simulink model "ssc_aircraft_elec_hybrid"  (R2025a)
settings: Solver=ode23t  StartTime=0.0  StopTime=FlightProfileLength  RelTol=1e-3  AbsTol=1e-3  EnableMultiTasking=on
PreLoadFcn:
  | ssc_aircraft_elec_default_params
PostLoadFcn:
  | warning('off','physmod:common:gl:sli:rtp:InvalidNonValueReference')
  | warning off Simulink:Engine:SortDiscontinuityInAlgLoop
model workspace (MATLAB code in the model file):
  | v0                 = 0; % Initial vehicle speed
  | wheel_radius = 0.15; % Wheel radius
  | k                   = 1e-2; % Motor losses (W/(N*M)^2)
  | t_torque        = 0.02; % Electric motor time constant
  | rpm0             = 2000; % Engine initial speed demand
undefined symbols (not defined in the file): Based, engine_ref_speed, gen_torque_demand, Height, motor_ref_speed
libraries: fl_lib x53, nesl_utility x31, ee_lib x9, ssc_aircraft_elec_lib x2, batteryecm_lib x1, simulink x1, sdl_lib x1, SimscapeFluids_lib x1
(part 1 of 2)
CloseFcn:
  | try,close(h1_ssc_aircraft_elec_hybrid),end
  | clear h1_ssc_aircraft_elec_hybrid
  | try,close(h2_ssc_aircraft_elec_hybrid),end
  | clear h2_ssc_aircraft_elec_hybrid
  | try,close(h3_ssc_aircraft_elec_hybrid),end
  | clear h3_ssc_aircraft_elec_hybrid
  | try,close(h4_ssc_aircraft_elec_hybrid),end
  | clear h4_ssc_aircraft_elec_hybrid
  | try,close(h5_ssc_aircraft_elec_hybrid),end
  | clear h5_ssc_aircraft_elec_hybrid
  | try,close(h6_ssc_aircraft_elec_hybrid),end
  | clear h6_ssc_aircraft_elec_hybrid
  | 
  | 
  | clear simlog_ssc_aircraft_elec_hybrid
  | clear logsout_ssc_aircraft_elec_hybrid
Description:
  | Hybrid Electric Aircraft Component Sizing
  | 
  | Copyright 2017-2025 The MathWorks, Inc.
settings Model: FPTRunName=Active  Creator=MathWorks  LastModifiedBy=smiller
settings SolverCC: AutoScaleAbsTol=off  AlgebraicLoopSolver=TrustRegion
settings DataIOCC: InitialState=xBaseline  LimitDataPoints=on  MaxDataPoints=10000  SaveOperatingPoint=on  SaveFormat=Array  ReturnWorkspaceOutputs=off  SignalLoggingName=simlog_ssc_aircraft_elec_hybrid
settings OptimizationCC: ReuseModelBlockBuffer=off  ExpressionDepthLimit=2147483647.0  LifeSpan=inf
settings DebuggingCC: AlgebraicLoopMsg=none  UnderspecifiedInitializationDetection=Classic  MergeDetectMultiDrivingBlocksExec=none  FcnCallInpInsideContextMsg=warning  UnconnectedInputMsg=warning  UnconnectedOutputMsg=warning  UnconnectedLineMsg=warning  StateNameClashWarn=warning  PregeneratedLibrarySubsystemCodeDiagnostic=none  SFUnexpectedBacktrackingDiag=warning  SFNoUnconditionalDefaultTransitionDiag=warning  SFExecutionAtInitializationDiag=none  ArithmeticOperatorsInVariantConditions=warning
settings HardwareCC: ProdBitPerPointer=32.0  ProdBitPerSizeT=32.0  ProdBitPerPtrDiffT=32.0  ProdLargestAtomicFloat=None  ProdIntDivRoundTo=Undefined  ProdEndianess=Unspecified  ProdWordSize=32.0  ProdHWDeviceType=32-bit Generic
settings ModelReferenceCC: EnableRefExpFcnMdlSchedulingChecks=on  PropagateSignalLabelsOutOfModel=off
settings SFSimCC: SimUseLocalCustomCode=off  CustomCodeUndefinedFunction=UseInterfaceOnly
settings RTWCC: RTWUseLocalCustomCode=off  GPUComputeCapability=3.5  DLArmComputeVersion=19.05
settings CodeAppCC: StateflowObjectComments=on
settings GRTTargetCC: TargetLangStandard=C89/C90 (ANSI)  CombineOutputUpdateFcns=off  GRTInterface=on
settings ConfigComp: CovMetricSettings=dw  CovSaveCumulativeToWorkspaceVar=on  CovSaveSingleToWorkspaceVar=on  CovExternalEMLEnable=off
settings SimscapeCC: SimscapeNormalizeSystem=off  SimscapeLogType=all  SimscapeLogSimulationStatistics=on  SimscapeLogName=simlog_ssc_aircraft_elec_hybrid  SimscapeLogDataHistory=10000.0

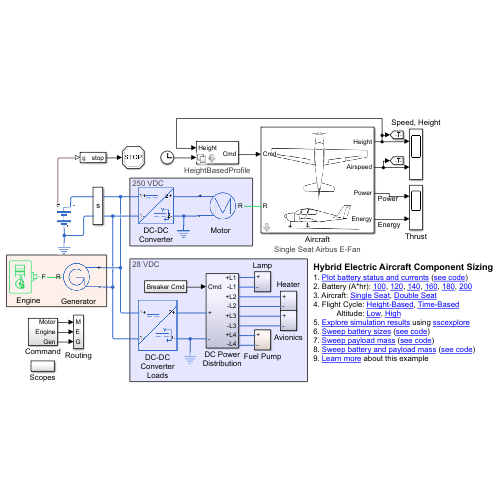
[thumbnail: Simulink's stored preview of the top-level diagram]
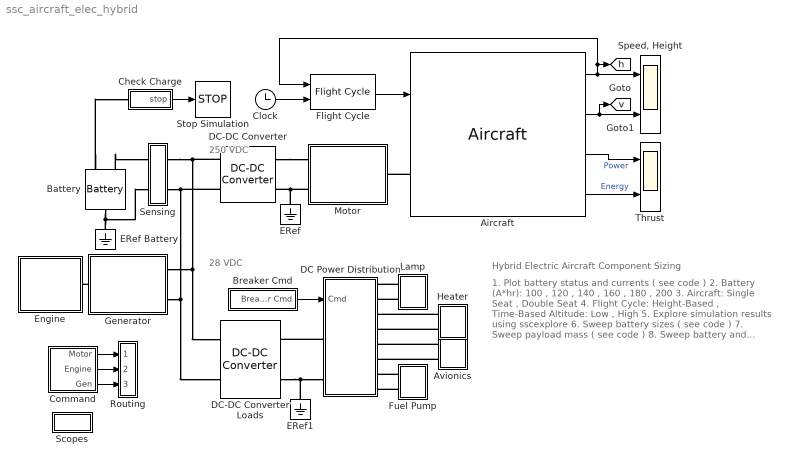
== system ssc_aircraft_elec_hybrid ==
  note: 250 VDC
  note: 28 VDC
  note: Hybrid Electric Aircraft Component Sizing
  note: 1. Plot battery status and currents ( see code )
      | 2. Battery (A*hr): 100 , 120 , 140 , 160 , 180 , 200
      | 3. Aircraft: Single Seat , Double Seat
      | 4. Flight Cycle: Height-Based , Time-Based
      | Altitude: Low , High
      | 5. Explore simulation results using sscexplore
      | 6. Sweep battery sizes ( see code )
      | 7. Sweep payload mass ( see code )
      | 8. Sweep battery and payload mass ( see code )
      | 9. Learn more about this example
  Aircraft : ssc_aircraft_elec_lib/Aircraft  Tag=PublishSubsystem  popup_aircraft_type=Single Seat Airbus E-Fan  aircraft_mass_cust=360  aircraft_wing_area_cust=10  aircraft_cl_cust=0.5  aircraft_cd_cust=0.05  battery_capacity=battery_capacity  battery_voltage=battery_vnom  battery_power_density=battery_pdensity  battery_mass=0  engine_system_mass=engine_system_mass  aircraft_max_thrust=max_thrust  aircraft_thrust_tau=thrust_tau  thrust_eff=thrust_eff  aircraft_h0=FlightProfileChoice.h0  aircraft_v0=0  earth_gravity=g_norm  checkbox_payload_mass=on  payload_mass=payload_mass
      settings: AttributesFormatString=%<popup_aircraft_type>
  Avionics : Subsystem
  Battery : batteryecm_lib/Battery  Vnom=201.6 V  prm_dir=1  R1_dis=2 Ohm  R1_ch=2 Ohm  R1=0.05 Ohm  prm_AH=2  AH=battery_capacity hr*A  V1=190 V  AH1=75 hr*A  prm_R2=1  R2=2000 Ohm  Tmeas=298.15 K  charge_measurement_port=simscape.enum.battery.enable.yes  prm_dyn=1  Rp1=0.005 Ohm  tau1=30 s  Rp2=0.005 Ohm  tau2=30 s  Rp3=0.005 Ohm  tau3=30 s  Rp4=0.005 Ohm  tau4=30 s  Rp5=0.005 Ohm  tau5=30 s  prm_fade=1  N_fade=100  AH_fade=45 hr*A  R1_fade=2.02 Ohm  R1_ch_fade=2.02 Ohm  V1_fade=10.35 V  prm_age=1  prm_age_OCV=1  OCV_age=0.9  SOC_age=60  Tmeas_age=298.15 K  delta_time_age_vec=[0] d  temperature_age_vec=[273] K  OCV_scaling_age=2.2134e6  OCV_offset_age=1.632e6  temp_exp_age=0.515833569 V  t_exp_age=0.75  Vnom_T2=12 V  R1_T2=2.2 Ohm  R1_T2_dis=2.2 Ohm  R1_T2_ch=2.2 Ohm  V1_T2=11.4 V  R2_T2=2200 Ohm  Rp1_T2=0.005 Ohm  tau1_T2=30 s  Rp2_T2=0.005 Ohm  tau2_T2=30 s  Rp3_T2=0.005 Ohm  tau3_T2=30 s  Rp4_T2=0.005 Ohm  tau4_T2=30 s  Rp5_T2=0.005 Ohm  tau5_T2=30 s  Tmeas2=273.15 K  thermal_port=simscape.enum.thermaleffects.omit  thermal_mass=30000 J/K  i_specify=off  i_priority=None  i=0 A  i_nominal_specify=off  i_nominal_value=1  i_nominal_unit=A  v_specify=off  v_priority=None  v=0 V  v_nominal_specify=off  v_nominal_value=1  v_nominal_unit=V  charge_specify=on  charge_priority=High  charge=battery_capacity hr*A  charge_nominal_specify=off  charge_nominal_value=1  charge_nominal_unit=A*hr  num_cycles_specify=off  num_cycles_priority=High  num_cycles=0  num_cycles_nominal_specify=off  num_cycles_nominal_value=1  num_cycles_nominal_unit=1  temperature_specify=off  temperature_priority=High  temperature=298.15 K  temperature_nominal_specify=off  temperature_nominal_value=1  temperature_nominal_unit=K
      settings: InternalSimscapePortConfiguration="{\"Bottom\":[],\"Left\":[{\"id\":\"p\",\"label\":\"+\",\"type\":\"foundation.electrical.electrical\"},{\"id\":\"q\",\"label\":\"q\",\"type\":\"output\"}],\"Right\":[{\"id\":\"n\",\"label\":\"-\",\"type\":\"foundation.electrical.electrical\"}],\"Top\":[]}"
  Breaker Cmd : Subsystem
  Check Charge : Subsystem  mask{q_battery_limit=20}
      mask prompts: q_battery_limit "Battery charge lower limit (A*hr)"
  Clock : Clock
  Command : Subsystem
  DC Power Distribution : Subsystem  Tag=PublishSubsystem
  DC-DC Converter : ee_lib/Semiconductors & Converters/Converters/DC-DC Converter  Vref_option=ee.enum.converters.voltageref.internal  v_ref=250 V  P_rated=200 kW  droop_enabled=true  droop_param=ee.enum.converters.droop.value  droop=0.001 V/A  droop_percent=2  Vref_droop=10 V  reversible=ee.enum.converters.directionality.bidirectional  G_diode=1e-8 1/Ohm  P_fixed=100 W  losses_option=ee.enum.converters.lossesOption.proportionalToSquaredCurrent  eff_rated=97  tableOption=ee.enum.converters.lossTableOption.current  i_eff_vec=[1, 2, 3, 4] A  v_eff_vec=[15, 30, 45] V  eff_vec=[90, 80, 70, 60]  eff_2D_table=[90, 85, 80; 80, 75, 70; 70, 65, 60; 60, 55, 50]  model_dynamics=ee.enum.converters.dynamics.yes  tau=0.02 s  v_ini=250 V  v1_min=1 V  R1=1000 Ohm  R2=1000 Ohm  fault_condition=ee.enum.faults.faultInputCondition.greaterThan  fault_threshold=0.5  T_eff_vec=[280, 300, 320] K  eff_3D_table=repmat([66; 76; 80; 74], 1, 3, 3)  thermal_mass=100 J/K  initial_temperature=298.15 K
      settings: InternalSimscapePortConfiguration="{\"Bottom\":[],\"Left\":[{\"id\":\"p1\",\"label\":\"1+\",\"type\":\"foundation.electrical.electrical\"},{\"id\":\"n1\",\"label\":\"1-\",\"type\":\"foundation.electrical.electrical\"}],\"Right\":[{\"id\":\"p2\",\"label\":\"2+\",\"type\":\"foundation.electrical.electrical\"},{\"id\":\"n2\",\"label\":\"2-\",\"type\":\"foundation.electrical.electrical\"}],\"Top\":[]}"
  DC-DC Converter Loads : ee_lib/Semiconductors & Converters/Converters/DC-DC Converter  Vref_option=ee.enum.converters.voltageref.internal  v_ref=28 V  P_rated=4 kW  droop_enabled=true  droop_param=ee.enum.converters.droop.value  droop=0.01 V/A  droop_percent=2  Vref_droop=10 V  reversible=ee.enum.converters.directionality.unidirectional  G_diode=1e-8 1/Ohm  P_fixed=100 W  losses_option=ee.enum.converters.lossesOption.proportionalToSquaredCurrent  eff_rated=97  tableOption=ee.enum.converters.lossTableOption.current  i_eff_vec=[1, 2, 3, 4] A  v_eff_vec=[15, 30, 45] V  eff_vec=[90, 80, 70, 60]  eff_2D_table=[90, 85, 80; 80, 75, 70; 70, 65, 60; 60, 55, 50]  model_dynamics=ee.enum.converters.dynamics.yes  tau=0.02 s  v_ini=28 V  v1_min=1 V  R1=1000 Ohm  R2=1000 Ohm  fault_condition=ee.enum.faults.faultInputCondition.greaterThan  fault_threshold=0.5  T_eff_vec=[280, 300, 320] K  eff_3D_table=repmat([66; 76; 80; 74], 1, 3, 3)  thermal_mass=100 J/K  initial_temperature=298.15 K
      settings: InternalSimscapePortConfiguration="{\"Bottom\":[],\"Left\":[{\"id\":\"p1\",\"label\":\"1+\",\"type\":\"foundation.electrical.electrical\"},{\"id\":\"n1\",\"label\":\"1-\",\"type\":\"foundation.electrical.electrical\"}],\"Right\":[{\"id\":\"p2\",\"label\":\"2+\",\"type\":\"foundation.electrical.electrical\"},{\"id\":\"n2\",\"label\":\"2-\",\"type\":\"foundation.electrical.electrical\"}],\"Top\":[]}"
  ERef : fl_lib/Electrical/Electrical Elements/Electrical Reference
  ERef Battery : fl_lib/Electrical/Electrical Elements/Electrical Reference
  ERef1 : fl_lib/Electrical/Electrical Elements/Electrical Reference
  Engine : Subsystem
      mask Display:
      | image('Driveline_Engine_IMAGE.png');
      | %{
      | patch([0 374 374 0 0],[183 40 40 183 183],[1 1 1]);
      | plot([200.294537656123;201.704177092068;202.879954177142;203.81054553527;204.486989062962;204.902770239264;205.053884864158;204.938877621199;204.558856093007;203.917480094638;203.02092642757;201.877829393721;200.499197642409;198.898308151034;197.090578360535;195.093417696999;192.926059909376;191.349221415216], [79.0962651705123;81.4129472419303;83.856642682368;86.4038173688741;89.0299406167901;91.7097214236537;94.4173520353776;97.1267564890293;99.8118417386092;102.446748945347;105.006102512455;107.465254465996;109.80052182835;111.989414698229;114.010852840726;115.845368701499;117.475294889959;118.468271604945])
      | plot([180.070315486255;177.215173525063;174.340173090774;171.473002009205;168.641272705228;165.872256280019;163.192619875453;160.628169854943;158.203603274058;155.942270034374;153.865948011161;151.994633320535;150.346347745932;148.936965178479;147.780058742747;146.886770080143;146.265702048809;145.922835873396;145.861473542603;146.08220600922;146.58290749893;147.358755982674;148.402279615432;149.703428694174;151.249672441989;153.026119686324;155.015662269112;157.199139807684;159.555524219735;162.062122235246;164.694793945081;167.42818528151;170.23597219174;173.091114152932;175.966114587221;178.83328566879;181.665014972767;184.434031397976;185.486929355725], [123.25590763568;123.598773811093;123.660136141886;123.439403675268;122.938702185559;122.162853701815;121.119330069056;119.818180990315;118.2719372425;116.495489998164;114.505947415377;112.322469876805;109.966085464754;107.459487449243;104.826815739408;102.093424402979;99.2856374927491;96.4304955315569;93.5554950972677;90.688324015699;87.8565947117214;85.0875782865128;82.4079418819464;79.8434918614364;77.4189252805513;75.1575920408679;73.081270017655;71.2099553270291;69.5616697524256;68.1522871849724;66.9953807492411;66.1020920866371;65.4810240553025;65.1381578798894;65.0767955490969;65.2975280157144;65.7982295054238;66.5740779891678;66.9481130562871])
      | plot([182.088349247351;182.056804583223;181.962474383197;181.806267098667;181.589687091173;181.314820144583;180.98431337785;180.601349751811;180.169617415534;179.693274187426;179.176907513169;178.625490286111;178.044332955585;177.439032384376;176.815417947876;176.17949539401;175.537389004603;174.895282615196;174.25936006133;173.63574562483;173.030445053621;172.449287723095;171.897870496037;171.38150382178;170.905160593672;170.473428257395;170.090464631356;169.759957864623;169.485090918033;169.268510910539;169.112303626009;169.017973425983;168.986428761855;169.017973425983;169.112303626009;169.268510910539;169.485090918033;169.759957864623;170.090464631356;170.473428257395;170.905160593672;171.38150382178;171.897870496037;172.449287723095;173.030445053621;173.63574562483;174.25936006133;174.895282615196;175.537389004603;176.17949539401;176.815417947876;177.439032384376;178.044332955585;178.625490286111;179.176907513169;179.693274187426;180.169617415534;180.601349751811;180.98431337785;181.314820144583;181.589687091173;181.806267098667;181.962474383197;182.056804583223;182.088349247351;182.088349247351], [94.3432759959251;93.7073437064164;93.0775357924916;92.4599176486499;91.8604372752408;91.2848679959696;90.7387528576339;90.2273512475527;89.7555882427917;89.3280071789786;88.9487258954975;88.6213970784445;88.3491730832641;88.1346755758426;87.9799702844327;87.8865471055612;87.8553057555109;87.8865471055612;87.9799702844327;88.1346755758426;88.3491730832641;88.6213970784445;88.9487258954975;89.3280071789786;89.7555882427917;90.2273512475527;90.7387528576339;91.2848679959696;91.8604372752408;92.4599176486499;93.0775357924916;93.7073437064164;94.3432759959251;94.9792082854337;95.6090161993586;96.2266343432003;96.8261147166093;97.4016839958805;97.9477991342162;98.4592007442974;98.9309637490584;99.3585448128716;99.7378260963527;100.065154913406;100.337378908586;100.551876416008;100.706581707417;100.800004886289;100.831246236339;100.800004886289;100.706581707417;100.551876416008;100.337378908586;100.065154913406;99.7378260963526;99.3585448128716;98.9309637490584;98.4592007442974;97.9477991342162;97.4016839958805;96.8261147166093;96.2266343432003;95.6090161993586;94.9792082854338;94.3432759959251;94.3432759959251])
      | plot([201.615249970928;201.583705306799;201.489375106774;201.333167822243;201.11658781475;200.84172086816;200.511214101427;200.128250475388;199.69651813911;199.220174911002;198.703808236745;198.152391009688;197.571233679162;196.965933107953;196.342318671452;195.706396117586;195.06428972818;194.422183338773;193.786260784907;193.162646348407;192.557345777197;191.976188446671;191.424771219614;190.908404545357;190.432061317249;190.000328980971;189.617365354932;189.286858588199;189.011991641609;188.795411634116;188.639204349585;188.54487414956;188.513329485431;188.54487414956;188.639204349585;188.795411634116;189.011991641609;189.286858588199;189.617365354932;190.000328980971;190.432061317249;190.908404545357;191.424771219614;191.976188446671;192.557345777197;193.162646348407;193.786260784907;194.422183338773;195.06428972818;195.706396117586;196.342318671452;196.965933107953;197.571233679162;198.152391009688;198.703808236745;199.220174911002;199.69651813911;200.128250475388;200.511214101427;200.84172086816;201.11658781475;201.333167822243;201.489375106774;201.583705306799;201.615249970928;201.615249970928], [74.7533852700144;74.1174529805057;73.487645066581;72.8700269227392;72.2705465493302;71.694977270059;71.1488621317233;70.6374605216421;70.165697516881;69.7381164530679;69.3588351695868;69.0315063525339;68.7592823573535;68.5447848499319;68.390079558522;68.2966563796505;68.2654150296003;68.2966563796505;68.390079558522;68.5447848499319;68.7592823573535;69.0315063525339;69.3588351695868;69.7381164530679;70.165697516881;70.6374605216421;71.1488621317233;71.694977270059;72.2705465493302;72.8700269227392;73.487645066581;74.1174529805057;74.7533852700144;75.3893175595231;76.0191254734479;76.6367436172896;77.2362239906986;77.8117932699698;78.3579084083055;78.8693100183867;79.3410730231478;79.7686540869609;80.147935370442;80.4752641874949;80.7474881826754;80.9619856900969;81.1166909815068;81.2101141603783;81.2413555104285;81.2101141603783;81.1166909815068;80.9619856900969;80.7474881826753;80.4752641874949;80.147935370442;79.7686540869609;79.3410730231478;78.8693100183867;78.3579084083055;77.8117932699698;77.2362239906986;76.6367436172896;76.0191254734479;75.3893175595231;74.7533852700145;74.7533852700144])
      | plot([201.615249970928;201.583705306799;201.489375106774;201.333167822243;201.11658781475;200.84172086816;200.511214101427;200.128250475388;199.69651813911;199.220174911002;198.703808236745;198.152391009688;197.571233679162;196.965933107953;196.342318671452;195.706396117586;195.06428972818;194.422183338773;193.786260784907;193.162646348407;192.557345777197;191.976188446671;191.424771219614;190.908404545357;190.432061317249;190.000328980971;189.617365354932;189.286858588199;189.011991641609;188.795411634116;188.639204349585;188.54487414956;188.513329485431;188.54487414956;188.639204349585;188.795411634116;189.011991641609;189.286858588199;189.617365354932;190.000328980971;190.432061317249;190.908404545357;191.424771219614;191.976188446671;192.557345777197;193.162646348407;193.786260784907;194.422183338773;195.06428972818;195.706396117586;196.342318671452;196.965933107953;197.571233679162;198.152391009688;198.703808236745;199.220174911002;199.69651813911;200.128250475388;200.511214101427;200.84172086816;201.11658781475;201.333167822243;201.489375106774;201.583705306799;201.615249970928;201.615249970928], [74.7533852700144;74.1174529805057;73.487645066581;72.8700269227392;72.2705465493302;71.694977270059;71.1488621317233;70.6374605216421;70.165697516881;69.7381164530679;69.3588351695868;69.0315063525339;68.7592823573535;68.5447848499319;68.390079558522;68.2966563796505;68.2654150296003;68.2966563796505;68.390079558522;68.5447848499319;68.7592823573535;69.0315063525339;69.3588351695868;69.7381164530679;70.165697516881;70.6374605216421;71.1488621317233;71.694977270059;72.2705465493302;72.8700269227392;73.487645066581;74.1174529805057;74.7533852700144;75.3893175595231;76.0191254734479;76.6367436172896;77.2362239906986;77.8117932699698;78.3579084083055;78.8693100183867;79.3410730231478;79.7686540869609;80.147935370442;80.4752641874949;80.7474881826754;80.9619856900969;81.1166909815068;81.2101141603783;81.2413555104285;81.2101141603783;81.1166909815068;80.9619856900969;80.7474881826753;80.4752641874949;80.147935370442;79.7686540869609;79.3410730231478;78.8693100183867;78.3579084083055;77.8117932699698;77.2362239906986;76.6367436172896;76.0191254734479;75.3893175595231;74.7533852700145;74.7533852700144])
      | plot([142.90856779553;142.90856779553;208.103220211342;208.103220211342], [139.948037685826;218.181620584801;218.181620584801;139.948037685826])
      | plot([142.90856779553;208.103220211342], [179.064829135314;179.064829135314])
      | plot([149.459528038278;149.459528038278], [179.064829135314;172.576858894899])
      | plot([201.615249970928;201.615249970928], [179.064829135314;172.576858894899])
      | plot([142.90856779553;208.103220211342;208.103220211342;142.90856779553;142.90856779553], [179.064829135314;179.064829135314;152.986968168989;152.986968168989;179.064829135314])
      | plot([142.90856779553;208.103220211342], [192.103759618476;192.103759618476])
      | plot([180.639579193667;200.229469919577], [99.0045361686498;79.4776354450732])
      | plot([173.332738922909;192.92262964882], [87.8553057555109;68.3284050319344])
      | plot([183.663099305704;200.481429928914], [153.553878189996;76.9580353517085])
      | plot([184.544959338382;174.970478983596], [95.0361660216004;153.553878189996])
      | plot([183.474129298702;186.749609420076;206.654450157657;201.615249970928;197.961829835549], [76.9580353517085;62.0923948008567;67.8874750155956;88.1702557671815;87.7923157531768])
      | plot([164.199188584462;187.694459455088], [94.7842060122639;95.1621460262686])
      | plot([175.537389004603;175.285428995267], [106.50034644641;81.9342455361038])
      | plot([142.90856779553;208.103220211342], [172.576858894899;172.576858894899])
      | plot([297.86397353746;317.389525743201], [71.0999651346356;71.0999651346356]+60)
      | plot([269.518472487107;297.86397353746;297.86397353746;269.518472487107;269.518472487107], [85.2727156598121;85.2727156598121;56.927214609459;56.927214609459;85.2727156598121]+60)
      | plot([258.180272066966;269.518472487107;269.518472487107;258.180272066966], [42.7544640842825;42.7544640842825;99.4454661849886;99.4454661849886]+60)
      | plot([108.893966535106;108.245686045801;107.603648851995;106.974038122836;106.362917353826;105.776171972045;105.219452656266;104.698120917834;104.217197466378;103.781313857637;103.394667889039;103.060983172626;102.783473274627;102.564810767061;102.40710148941;102.31186426823;102.280016290024;102.280016290024;102.31186426823;102.40710148941;102.564810767061;102.783473274627;103.060983172626;103.394667889039;103.781313857637;104.217197466378;104.698120917834;105.219452656266;105.776171972045;106.362917353826;106.974038122836;107.603648851995;108.245686045801;108.893966535106;249.67662175186;250.324902241165;250.966939434972;251.596550164131;252.20767093314;252.794416314921;253.3511356307;253.872467369133;254.353390820588;254.78927442933;255.175920397927;255.50960511434;255.787115012339;256.005777519905;256.163486797556;256.258724018736;256.290571996942;256.290571996942;256.258724018736;256.163486797556;256.005777519905;255.787115012339;255.50960511434;255.175920397927;254.78927442933;254.353390820588;253.872467369133;253.3511356307;252.794416314921;252.20767093314;251.596550164131;250.966939434972;250.324902241165;249.67662175186;108.893966535106], [233.173241140321;233.141393162114;233.046155940935;232.888446663284;232.669784155718;232.392274257719;232.058589541306;231.671943572708;231.236059963967;230.755136512511;230.233804774079;229.6770854583;229.090340076519;228.479219307509;227.84960857835;227.207571384544;226.559290895239;46.5338642243296;45.8855837350246;45.2435465412178;44.6139358120588;44.0028150430496;43.4160696612682;42.8593503454891;42.3380186070568;41.8570951556014;41.4212115468599;41.0345655782626;40.7008808618494;40.42337096385;40.2047084562844;40.0469991786335;39.9517619574538;39.9199139792472;39.9199139792472;39.9517619574538;40.0469991786335;40.2047084562844;40.42337096385;40.7008808618494;41.0345655782626;41.4212115468599;41.8570951556014;42.3380186070568;42.8593503454891;43.4160696612682;44.0028150430496;44.6139358120588;45.2435465412178;45.8855837350246;46.5338642243296;226.559290895239;227.207571384544;227.84960857835;228.479219307509;229.090340076519;229.6770854583;230.233804774079;230.755136512511;231.236059963967;231.671943572708;232.058589541306;232.392274257719;232.669784155718;232.888446663284;233.046155940935;233.141393162114;233.173241140321;233.173241140321])
      | %}
  Flight Cycle : ssc_aircraft_elec_lib/Flight Cycle  popup_flight_cycle_type=Height-Based  flight_cycle_max_height=FlightProfileChoice.FlightProfileHeight  flight_cycle_ascent_start_time=FlightProfileChoice.LevelFlightTime  flight_cycle_duration=FlightProfileChoice.FlightProfileLength  flight_cycle_ascent_duration=FlightProfileChoice.ClimbFlightTime
      settings: AttributesFormatString=%<ActiveVariant>
  Fuel Pump : Subsystem  Tag=PublishSubsystem
  Generator : Subsystem  Tag=PublishSubsystem
      mask Display:
      | image('Generator_IMAGE.png');
      | % Circle
      | %{
      | plot(sin(0:0.1:2.2*pi)*0.9,cos(0:0.1:2.2*pi)*0.9);
      | 
      | % In/out
      | plot([-1.5 -0.9],[0 0]);
      | plot([1.5 0.58],[1 1]*0.65);
      | plot([1.5 0.55],-[1 1]*0.68);
      | 
      | % 'M'
      | %plot([0.5 0.5],[-0.5 0.5]);
      | %plot([-0.5 -0.5],[-0.5 0.5]);
      | %plot([0.5 0],[0.5 -0.5]);
      | %plot([-0.5 0],[0.5 -0.5]);
      | 
      | % 'G'
      | plot(sin(0.5:-0.1:-1.5*pi)*0.5,cos(-0.5:0.1:1.5*pi)*0.5);
      | plot([0 0.5 0.5],[0 0 -0.5]);
      | 
      | % Plot points to set plot range
      | color('white');plot(1.9,1.2);plot(-1.9,-1.2)
      | color('black');
      | %}
  Heater : Subsystem
  Lamp : Subsystem
  Motor : Subsystem  Tag=PublishSubsystem
      mask Display: image('Motor_IMAGE.png');
  Routing : Subsystem
  Scopes : Subsystem
  Sensing : Subsystem
      mask Display: disp('s');
  "Speed, Height" : Scope  NumInputPorts=2
      settings: ActiveDisplayYMinimum=-12.5  ActiveDisplayYMaximum=1112.5
  Stop Simulation : Stop
  Thrust : Scope  NumInputPorts=2
      settings: ActiveDisplayYMinimum=13.58364  ActiveDisplayYMaximum=68.87509  DataLoggingMaxPoints=50000  DataLoggingVariableName=ScopeData6
  tag scope: h=global, v=global
  wires:
  Command/1(Motor) -> Routing/1(M)
  Aircraft/2 -> [v], "Speed, Height"/2
  Aircraft/3 -> Thrust/1  "Power"
  Aircraft/4 -> Thrust/2  "Energy"
  Command/2(Engine) -> Routing/2(E)
  Command/3(Gen) -> Routing/3(G)
  Clock/1 -> Flight Cycle/2
  Aircraft/1 -> [h], Flight Cycle/1, "Speed, Height"/1
  Flight Cycle/1 -> Aircraft/1
  Check Charge/1(stop) -> Stop Simulation/1
  Breaker Cmd/1(Breaker Cmd) -> DC Power Distribution/1(Cmd)
  connections:
  Aircraft/LConn1 -- Motor/LConn1
  DC-DC Converter/RConn1 -- Motor/RConn1
  DC Power Distribution/LConn1 -- DC-DC Converter Loads/RConn1
  Heater/LConn1 -- DC Power Distribution/RConn3
  Lamp/LConn2 -- DC Power Distribution/RConn2
  Lamp/LConn1 -- DC Power Distribution/RConn1
  Heater/LConn2 -- DC Power Distribution/RConn4
  DC-DC Converter Loads/RConn2 -- DC Power Distribution/LConn2 -- ERef1/LConn1
  ERef/LConn1 -- Motor/RConn2 -- DC-DC Converter/RConn2
  DC-DC Converter/LConn1 -- Generator/RConn1 -- DC-DC Converter Loads/LConn1 -- Sensing/RConn1
  Sensing/RConn2 -- DC-DC Converter/LConn2 -- Generator/RConn2 -- DC-DC Converter Loads/LConn2
  Avionics/LConn1 -- DC Power Distribution/RConn5
  Avionics/LConn2 -- DC Power Distribution/RConn6
  Generator/LConn1 -- Engine/RConn1
  Fuel Pump/LConn1 -- DC Power Distribution/RConn7
  Fuel Pump/LConn2 -- DC Power Distribution/RConn8
  Battery/LConn2 -- Check Charge/LConn1
  Battery/LConn1 -- Sensing/LConn1
  Battery/RConn1 -- ERef Battery/LConn1 -- Sensing/LConn2

== system ssc_aircraft_elec_hybrid/Avionics ==
  Electrical Power : Subsystem
  Resistor : fl_lib/Electrical/Electrical Elements/Resistor  R=1.5 Ohm  i_specify=off  i_priority=None  i=0 A  i_nominal_specify=off  i_nominal_value=1  i_nominal_unit=A  v_specify=off  v_priority=None  v=0 V  v_nominal_specify=off  v_nominal_value=1  v_nominal_unit=V
  + : PMIOPort  Side=Left
  - : PMIOPort  Port=2  Side=Left
  connections:
  Electrical Power/LConn1 -- +/RConn1
  Resistor/LConn1 -- Electrical Power/RConn1
  Electrical Power/LConn2 -- Resistor/RConn1 -- -/RConn1

== system ssc_aircraft_elec_hybrid/Breaker Cmd ==
  Avionics Breaker : Constant
  Fuel Pump Breaker : Constant
  Heater Breaker OFF : Constant  Value=0
  Heater Breaker ON : Constant
  Lamp Breaker : Constant
  Mux : Mux
  Switch : Switch  Threshold=800  SaturateOnIntegerOverflow=off  InputSameDT=off
  Breaker Cmd : Outport  VectorParamsAs1DForOutWhenUnconnected=off
  wires:
  Fuel Pump Breaker/1 -> Mux/4
  Lamp Breaker/1 -> Mux/1
  Avionics Breaker/1 -> Mux/3
  Switch/1 -> Mux/2
  Mux/1 -> Breaker Cmd/1
  Heater Breaker OFF/1 -> Switch/3
  [h] -> Switch/2
  Heater Breaker ON/1 -> Switch/1

== system ssc_aircraft_elec_hybrid/Check Charge ==
  Compare To Constant : simulink/Logic and Bit Operations/Compare To Constant  relop=<=  const=q_battery_limit  OutDataTypeStr=boolean
  PS-Simulink Converter : nesl_utility/PS-Simulink Converter  PhysicalDomain=network_engine_domain  SubClassName=ps_output  LeftPortType=input  RightPortType=output  PseudoPeriodic=off  Frequencies=[]  VectorFormat=1-D array  Unit=A*hr  AffineConversion=off
  q : PMIOPort  Side=Left
  stop : Outport  VectorParamsAs1DForOutWhenUnconnected=off
  tag scope: Chg_battery=global
  wires:
  PS-Simulink Converter/1 -> [Chg_battery], Compare To Constant/1
  Compare To Constant/1 -> stop/1
  connections:
  q/RConn1 -- PS-Simulink Converter/LConn1

== system ssc_aircraft_elec_hybrid/Command ==
  Engine RPM demand : Constant  Value=engine_ref_speed
  Gain : Gain  Gain=-1
  Generator torque demand : Constant  Value=gen_torque_demand
  Ref RPM : Constant  Value=motor_ref_speed
  Steady-state correction factor as proportional-only control : Gain  Gain=1.08
  Motor : Outport  VectorParamsAs1DForOutWhenUnconnected=off
  Engine : Outport  Port=2  VectorParamsAs1DForOutWhenUnconnected=off
  Gen : Outport  Port=3  VectorParamsAs1DForOutWhenUnconnected=off
  wires:
  Ref RPM/1 -> Motor/1
  Generator torque demand/1 -> Gain/1
  Steady-state correction factor as proportional-only control/1 -> Engine/1
  Engine RPM demand/1 -> Steady-state correction factor as proportional-only control/1
  Gain/1 -> Gen/1

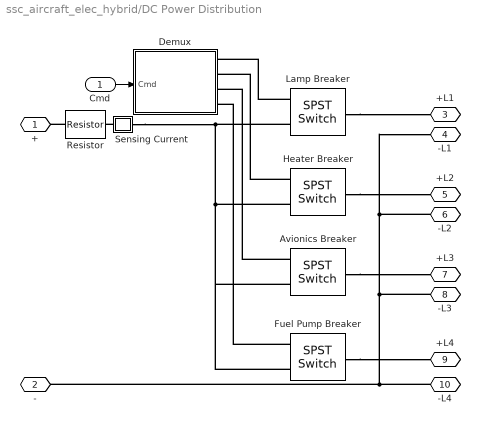
== system ssc_aircraft_elec_hybrid/DC Power Distribution ==
  Cmd : Inport
  Avionics Breaker : ee_lib/Switches & Breakers/SPST Switch  R_closed=0.001 Ohm  G_open=1e-3 S  Threshold=0.5 V  Width=0 V  model_dynamics=0  t_on=1e-3 s  t_off=1e-3 s  initial_vT=0 V
      settings: InternalSimscapePortConfiguration="{\"Bottom\":[],\"Left\":[{\"id\":\"vT\",\"label\":\"vT\",\"type\":\"input\"},{\"id\":\"p\",\"label\":\"\",\"type\":\"foundation.electrical.electrical\"}],\"Right\":[{\"id\":\"n\",\"label\":\"\",\"type\":\"foundation.electrical.electrical\"}],\"Top\":[]}"
  Demux : Subsystem
  Fuel Pump Breaker : ee_lib/Switches & Breakers/SPST Switch  R_closed=0.001 Ohm  G_open=1e-3 S  Threshold=0.5 V  Width=0 V  model_dynamics=0  t_on=1e-3 s  t_off=1e-3 s  initial_vT=0 V
      settings: InternalSimscapePortConfiguration="{\"Bottom\":[],\"Left\":[{\"id\":\"vT\",\"label\":\"vT\",\"type\":\"input\"},{\"id\":\"p\",\"label\":\"\",\"type\":\"foundation.electrical.electrical\"}],\"Right\":[{\"id\":\"n\",\"label\":\"\",\"type\":\"foundation.electrical.electrical\"}],\"Top\":[]}"
  Heater Breaker : ee_lib/Switches & Breakers/SPST Switch  R_closed=0.001 Ohm  G_open=1e-3 S  Threshold=0.5 V  Width=0 V  model_dynamics=0  t_on=1e-3 s  t_off=1e-3 s  initial_vT=0 V
      settings: InternalSimscapePortConfiguration="{\"Bottom\":[],\"Left\":[{\"id\":\"vT\",\"label\":\"vT\",\"type\":\"input\"},{\"id\":\"p\",\"label\":\"\",\"type\":\"foundation.electrical.electrical\"}],\"Right\":[{\"id\":\"n\",\"label\":\"\",\"type\":\"foundation.electrical.electrical\"}],\"Top\":[]}"
  Lamp Breaker : ee_lib/Switches & Breakers/SPST Switch  R_closed=0.001 Ohm  G_open=1e-3 S  Threshold=0.5 V  Width=0 V  model_dynamics=0  t_on=1e-3 s  t_off=1e-3 s  initial_vT=0 V
      settings: InternalSimscapePortConfiguration="{\"Bottom\":[],\"Left\":[{\"id\":\"vT\",\"label\":\"vT\",\"type\":\"input\"},{\"id\":\"p\",\"label\":\"\",\"type\":\"foundation.electrical.electrical\"}],\"Right\":[{\"id\":\"n\",\"label\":\"\",\"type\":\"foundation.electrical.electrical\"}],\"Top\":[]}"
  Resistor : fl_lib/Electrical/Electrical Elements/Resistor  R=0.002 Ohm  i_specify=off  i_priority=None  i=0 A  i_nominal_specify=off  i_nominal_value=1  i_nominal_unit=A  v_specify=off  v_priority=None  v=0 V  v_nominal_specify=off  v_nominal_value=1  v_nominal_unit=V
  Sensing Current : Subsystem
      mask Display: disp('i')
  + : PMIOPort  Side=Left
  - : PMIOPort  Port=2  Side=Left
  +L1 : PMIOPort  Port=3  Side=Right
  -L1 : PMIOPort  Port=4  Side=Right
  +L2 : PMIOPort  Port=5  Side=Right
  -L2 : PMIOPort  Port=6  Side=Right
  +L3 : PMIOPort  Port=7  Side=Right
  -L3 : PMIOPort  Port=8  Side=Right
  +L4 : PMIOPort  Port=9  Side=Right
  -L4 : PMIOPort  Port=10  Side=Right
  wires:
  Cmd/1 -> Demux/1(Cmd)
  connections:
  -L4/RConn1 -- -L1/RConn1 -- -L2/RConn1 -- -L3/RConn1 -- -/RConn1
  Lamp Breaker/RConn1 -- +L1/RConn1
  Heater Breaker/RConn1 -- +L2/RConn1
  Avionics Breaker/RConn1 -- +L3/RConn1
  Fuel Pump Breaker/RConn1 -- +L4/RConn1
  Resistor/LConn1 -- +/RConn1
  Lamp Breaker/LConn1 -- Demux/RConn1
  Heater Breaker/LConn1 -- Demux/RConn2
  Avionics Breaker/LConn1 -- Demux/RConn3
  Fuel Pump Breaker/LConn1 -- Demux/RConn4
  Fuel Pump Breaker/LConn2 -- Avionics Breaker/LConn2 -- Heater Breaker/LConn2 -- Lamp Breaker/LConn2 -- Sensing Current/RConn1
  Sensing Current/LConn1 -- Resistor/RConn1

== system ssc_aircraft_elec_hybrid/Engine ==
  Engine : sdl_lib/Engines & Motors/Generic Engine  input_type=sdl.enum.GenericEngineInputType.NormalizedThrottle  model_parameterization=1  engine_type=1  Trq_max=380 N*m  w_Trq_max=4300 rpm  P_max=50e3 W  w_P_max=5500 rpm  w_max=7000 rpm  w_min=500 rpm  w_tab=[ 500 1000 2e+3 3e+3 4e+3 5e+3 6e+3 7e+3 ] rpm  trq_tab=[ 380 380 380 380 350 280 200 80 ] N*m  pwr_tab=[ 2e+4 4e+4 7.8e+4 1.2e+5 1.45e+5 1.48e+5 1.25e+5 6e+4 ] W  interp_method=1  w_thr=20 rpm  model_inertia=1  inertia=0.2 kg*m^2  initial_velocity=2000 rpm  model_time_constant=1  time_constant=0.2 s  initial_normalized_throttle=0.15  fc_model=4  fc_per_rev=25 mg/rev  fc_w_tab=[ 1000 2e+3 3e+3 4e+3 5e+3 6e+3 ] rpm  fc_trq_tab=[ 0 80 160 200 240 320 360 400 ] N*m  fc_tab=[ 0.5 0.9 1.4 1.6 1.9 2.7 3.4 4.4; 1 1.7 2.7 3.1 3.6 5 6 7.4; 1.4 2.7 4 4.8 5.6 7.5 8.5 10.5; 2 3.6 5.8 6.7 8 10.4 11.7 13.3; 2.5 4.8 7.9 9.4 10.8 14 16.2 18.6; 3.1 6 10.3 11.9 13.8 18.4 22 26.5 ] g/s  bmep_tab=[ 0 250 500 625 750 1000 1.15e+3 1.25e+3 ] kPa  bsfc_tab=[ 410 380 300 280 270 290 320 380; 410 370 290 270 260 270 285 320; 415 380 290 275 265 270 270 300; 420 390 310 290 285 280 280 285; 430 410 340 320 310 300 310 320; 450 430 370 340 330 330 350 380 ] g/hr/kW  fc_interp_method=1  displaced_volume=400 cm^3  rev_per_cycle=2  idle_speed=0  idle_speed_reference=1000 rpm  tau_controller=1 s  idle_w_thr=1 rpm  redline=0  redline_speed=5000 rpm  tau_redline=1 s  redline_w_thr=1 rpm
      settings: InternalSimscapePortConfiguration="{\"Bottom\":[],\"Left\":[{\"id\":\"ThrNorm\",\"label\":\"Thr\",\"type\":\"input\"},{\"id\":\"B\",\"label\":\"B\",\"type\":\"foundation.mechanical.rotational.rotational\"}],\"Right\":[{\"id\":\"P\",\"label\":\"P\",\"type\":\"output\"},{\"id\":\"FC\",\"label\":\"FC\",\"type\":\"output\"},{\"id\":\"F\",\"label\":\"F\",\"type\":\"foundation.mechanical.rotational.rotational\"}],\"Top\":[]}"
  Engine Management : Subsystem
  RPM Sensor : Subsystem
      mask Display: disp('S');
  Reference : fl_lib/Mechanical/Rotational Elements/Mechanical Rotational Reference
  Sensor Fuel : Subsystem
  Sensor Power : Subsystem
  Simulink-PS Converter : nesl_utility/Simulink-PS Converter  PhysicalDomain=network_engine_domain  SubClassName=ps_input  LeftPortType=input  RightPortType=output  PseudoPeriodic=off  Frequencies=[]  NoiseDistribution=none  NoiseParameters=[]  Unit=1  AffineConversion=off  FilteringAndDerivatives=zero  SimscapeFilterOrder=1  InputFilterTimeConstant=.001  UdotUserProvided=0
  F : PMIOPort  Side=Right
  wires:
  RPM Sensor/1(rpm) -> Engine Management/2(rpm)
  [ref_engine_speed] -> Engine Management/1(rpm_dem)
  Engine Management/1(T) -> Simulink-PS Converter/1
  connections:
  F/RConn1 -- Engine/RConn3 -- RPM Sensor/LConn1
  Reference/LConn1 -- Engine/LConn2
  Simulink-PS Converter/RConn1 -- Engine/LConn1
  Engine/RConn1 -- Sensor Power/LConn1
  Engine/RConn2 -- Sensor Fuel/LConn1

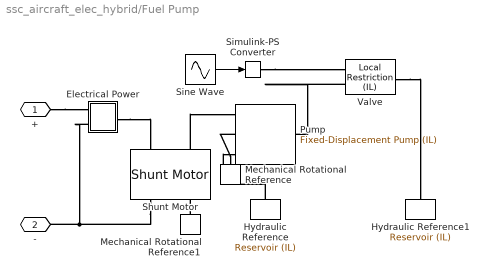
== system ssc_aircraft_elec_hybrid/Fuel Pump ==
  Electrical Power : Subsystem
  Hydraulic Reference : fl_lib/Isothermal Liquid/Elements/Reservoir (IL)  reservoir_type=foundation.enum.constant_controlled.constant  pressure_spec=foundation.enum.pressure_spec.atmospheric  reservoir_pressure=0.101325 MPa
  Hydraulic Reference1 : fl_lib/Isothermal Liquid/Elements/Reservoir (IL)  reservoir_type=foundation.enum.constant_controlled.constant  pressure_spec=foundation.enum.pressure_spec.atmospheric  reservoir_pressure=0.101325 MPa
  Mechanical Rotational Reference1 : fl_lib/Mechanical/Rotational Elements/Mechanical Rotational Reference
  Mechanical Rotational Reference : fl_lib/Mechanical/Rotational Elements/Mechanical Rotational Reference
  Pump : SimscapeFluids_lib/Isothermal Liquid/Pumps & Motors/Fixed-Displacement Pump (IL)  leakage_friction_spec=fluids.isothermal_liquid.pumps_motors.enum.pump_motor_loss_spec.analytical  displacement=5e-6 m^3/rad  omega_nominal=188 rad/s  p_nominal=100e5 Pa  vol_eff_nominal=0.92  mech_eff_nominal=0.8695652173913044  no_load_torque=0 N*m  p_diff_eff_TLU=[100000.0, 1000000.0, 2000000.0] Pa  omega_eff_TLU=[25.0, 50.0, 100.0, 200.0, 300.0, 400.0] rad/s  vol_eff_TLU=[0.816, 0.908, 0.954, 0.977, 0.981, 0.984; 0.325, 0.663, 0.831, 0.916, 0.925, 0.946; 0.137, 0.568, 0.78, 0.892, 0.893, 0.91]  mech_eff_TLU=[0.996, 0.996, 0.996, 0.996, 0.996, 0.996; 0.988, 0.989, 0.989, 0.989, 0.989, 0.99; 0.981, 0.981, 0.982, 0.982, 0.983, 0.984]  p_diff_loss_TLU=[100000.0, 1000000.0, 2000000.0] Pa  omega_loss_TLU=[25.0, 50.0, 100.0, 200.0, 300.0, 400.0] rad/s  vol_loss_TLU=[0.023, 0.023, 0.023, 0.023, 0.0285, 0.032; 0.0844, 0.0842, 0.0845, 0.084, 0.1125, 0.108; 0.1079, 0.108, 0.11, 0.108, 0.1605, 0.18] * 1e-3 m^3/s  mech_loss_TLU=[0.002, 0.002, 0.002, 0.002, 0.002, 0.002; 0.0607, 0.0556, 0.0556, 0.0556, 0.0556, 0.0505; 0.1937, 0.1937, 0.1833, 0.1833, 0.1729, 0.1626] N*m  vol_eff_min=1e-3  vol_eff_max=1  mech_eff_min=1e-3  mech_eff_max=1  pressure_threshold=1e5 Pa  omega_threshold=10 rad/s  supplied_range_check=simscape.enum.assert.action.none  pump_mode_check=simscape.enum.assert.action.none  pressure_check=simscape.enum.assert.action.none  p_min_valid=0 + 101325 Pa
      settings: LibrarySourceBlock=SimscapeFluids_lib/Isothermal Liquid/Pumps & Motors/Fixed-Displacement Pump (IL)  InternalSimscapePortConfiguration="{\"Bottom\":[{\"id\":\"A\",\"label\":\"A\",\"type\":\"foundation.isothermal_liquid.isothermal_liquid\"}],\"Left\":[],\"Right\":[{\"id\":\"R\",\"label\":\"R\",\"type\":\"foundation.mechanical.rotational.rotational\"},{\"id\":\"C\",\"label\":\"C\",\"type\":\"foundation.mechanical.rotational.rotational\"}],\"Top\":[{\"id\":\"B\",\"label\":\"B\",\"type\":\"foundation.isothermal_liquid.isothermal_liquid\"}]}"
  Shunt Motor : ee_lib/Electromechanical/Brushed Motors/Shunt Motor  parameterization=1  Ra=0.35 Ohm  Rf=240 Ohm  Laf=1 s*V/rad/A  w_max=4.6e+3 rpm  w_rated=4e+3 rpm  P_rated=50 W  V_rated=220 V  I_start=2.09 A  La=1e-4 H  Lf=12 H  J=0.0005 kg*m^2  lam=1.5/200 N*m/(rad/s)  speed0=0 rpm  i_a_specify=off  i_a_priority=None  i_a=0 A  i_a_nominal_specify=off  i_a_nominal_value=1  i_a_nominal_unit=A  i_f_specify=off  i_f_priority=None  i_f=0 A  i_f_nominal_specify=off  i_f_nominal_value=1  i_f_nominal_unit=A  alpha=[.00393, .00393] 1/K  Tmeas=25 degC  thermal_masses=[100, 100] J/K  initial_temperatures=[25, 25] degC
      settings: InternalSimscapePortConfiguration="{\"Bottom\":[],\"Left\":[{\"id\":\"p\",\"label\":\"+\",\"type\":\"foundation.electrical.electrical\"},{\"id\":\"R\",\"label\":\"R\",\"type\":\"foundation.mechanical.rotational.rotational\"}],\"Right\":[{\"id\":\"n\",\"label\":\"-\",\"type\":\"foundation.electrical.electrical\"},{\"id\":\"C\",\"label\":\"C\",\"type\":\"foundation.mechanical.rotational.rotational\"}],\"Top\":[]}"
  Simulink-PS Converter : nesl_utility/Simulink-PS Converter  PhysicalDomain=network_engine_domain  SubClassName=ps_input  LeftPortType=input  RightPortType=output  PseudoPeriodic=off  Frequencies=[]  NoiseDistribution=none  NoiseParameters=[]  Unit=1  AffineConversion=off  FilteringAndDerivatives=zero  SimscapeFilterOrder=1  InputFilterTimeConstant=0.001  UdotUserProvided=1
  Sine Wave : Sin  Amplitude=1e-4  Bias=1e-3  Frequency=2  SampleTime=0
  Valve : fl_lib/Isothermal Liquid/Elements/Local Restriction (IL)  restriction_type=foundation.enum.restriction_type.variable  restriction_area=1e-3 m^2  min_area=1e-12 m^2  max_area=1e10 m^2  area=inf m^2  Cd=0.7  Re_c=12  pressure_recovery=false
      settings: LibrarySourceBlock=fl_lib/Isothermal Liquid/Elements/Local Restriction (IL)  InternalSimscapePortConfiguration="{\"Bottom\":[],\"Left\":[{\"id\":\"A\",\"label\":\"A\",\"type\":\"foundation.isothermal_liquid.isothermal_liquid\"},{\"id\":\"AR\",\"label\":\"AR\",\"type\":\"input\"}],\"Right\":[{\"id\":\"B\",\"label\":\"B\",\"type\":\"foundation.isothermal_liquid.isothermal_liquid\"}],\"Top\":[]}"
  + : PMIOPort  Side=Left
  - : PMIOPort  Port=2  Side=Left
  wires:
  Sine Wave/1 -> Simulink-PS Converter/1
  connections:
  Shunt Motor/RConn1 -- Electrical Power/LConn2 -- -/RConn1
  Electrical Power/RConn1 -- Shunt Motor/LConn1
  Mechanical Rotational Reference1/LConn1 -- Shunt Motor/RConn2
  +/RConn1 -- Electrical Power/LConn1
  Pump/RConn2 -- Mechanical Rotational Reference/LConn1
  Valve/RConn1 -- Hydraulic Reference1/LConn1
  Simulink-PS Converter/RConn1 -- Valve/LConn2
  Hydraulic Reference/LConn1 -- Pump/RConn3
  Valve/LConn1 -- Pump/LConn1
  Shunt Motor/LConn2 -- Pump/RConn1

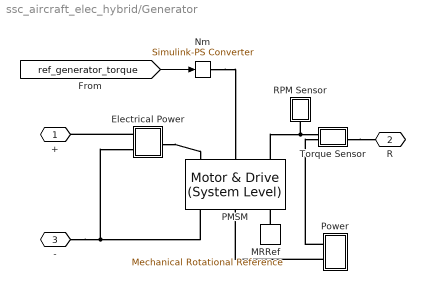
== system ssc_aircraft_elec_hybrid/Generator ==
  Electrical Power : Subsystem
  MRRef : fl_lib/Mechanical/Rotational Elements/Mechanical Rotational Reference
  Nm : nesl_utility/Simulink-PS Converter  PhysicalDomain=network_engine_domain  SubClassName=ps_input  LeftPortType=input  RightPortType=output  PseudoPeriodic=off  Frequencies=[]  NoiseDistribution=none  NoiseParameters=[]  Unit=N*m  AffineConversion=off  FilteringAndDerivatives=zero  SimscapeFilterOrder=1  InputFilterTimeConstant=.001  UdotUserProvided=1
  PMSM : ee_lib/Electromechanical/Motor & Drive (System Level)  torque_speed_param=1  overtorque_param=ee.enum.electromech.overtorque.no  T_t=[ 0.9 0.8 0.7 0 ]*500 N*m  T_t_intermittent=[.36, .32, .28, 0] N*m  T_t_2D=[.09, .09, .09; .08, .08, .08; .07, .07, .07; 0, 0, 0] N*m  T_t_intermittent_2D=[.36, .36, .36; .32, .32, .32; .28, .28, .28; 0, 0, 0] N*m  w_t=[ 0 3.75e+3 7.5e+3 8e+3 ] rpm  vdc_t=[6, 12, 24] V  torque_max=0.1 N*m  power_max=30 W  torque_max_intermittent=0.4 N*m  power_max_intermittent=120 W  time_overtorque=30 s  time_recover=60 s  Tc=0.02 s  EnableSwitch=simscape.enum.onoff.off  losses_param=1  eff=95  w_eff=3.75e+3 rpm  T_eff=400 N*m  Piron=0 W  Pbase=0 W  w_eff_vec=[-8000 -4000 0 4000 8000] rpm  T_eff_vec=[0 0.03 0.06 0.09] N*m  v_eff_vec=[100, 250, 400] V  losses_mat=[1.49 1.67 2.21 3.10; 0.42 0.69 1.14 2.03; 0.06 0.24 0.78 1.68; 0.42 0.69 1.14 2.03; 1.49 1.67 2.21 3.10] W  efficiency_mat=[95 95 95 95; 95 95 95 95; 95 95 95 95; 95 95 95 95; 95 95 95 95]  losses_mat_3D=ones(5, 4, 3) W  efficiency_mat_3D=95 * ones(5, 4, 3)  Res=0 Ohm  J=0 kg*m^2  lam=1e-5 N*m/(rad/s)  speed0=0 rpm  faulted_specify=off  faulted_priority=None  faulted=0  faulted_nominal_specify=off  faulted_nominal_value=1  faulted_nominal_unit=1  isSwitchedOff_specify=off  isSwitchedOff_priority=None  isSwitchedOff=0  isSwitchedOff_nominal_specify=off  isSwitchedOff_nominal_value=1  isSwitchedOff_nominal_unit=1  torqueLimitContinuous_specify=off  torqueLimitContinuous_priority=None  torqueLimitContinuous=0 N*m  torqueLimitContinuous_nominal_specify=off  torqueLimitContinuous_nominal_value=1  torqueLimitContinuous_nominal_unit=N*m  alpha=3.93e-3 1/K  Tmeas=25 degC  Tmeas2=125 degC  losses_mat_T2=[1.49, 1.74, 2.49, 3.74; .42, .67, 1.42, 2.67; .06, .31, 1.06, 2.31; .42, .67, 1.42, 2.67; 1.49, 1.74, 2.49, 3.74] W  efficiency_mat_T2=[95, 95, 95, 95; 95, 95, 95, 95; 95, 95, 95, 95; 95, 95, 95, 95; 95, 95, 95, 95]  losses_mat_3D_T2=ones(5, 4, 3) W  efficiency_mat_3D_T2=95 * ones(5, 4, 3)  thermal_mass=100 J/K  initial_temperature=25 degC
  Power : Subsystem
  RPM Sensor : Subsystem
      mask Display: disp('w')
  Torque Sensor : Subsystem
      mask Display: disp('trq')
  + : PMIOPort  Side=Right
  R : PMIOPort  Port=2  Side=Left
  - : PMIOPort  Port=3  Side=Right
  wires:
  [ref_generator_torque] -> Nm/1
  connections:
  Nm/RConn1 -- PMSM/LConn2
  PMSM/LConn3 -- Torque Sensor/LConn1 -- RPM Sensor/LConn1
  MRRef/LConn1 -- PMSM/RConn3
  Electrical Power/RConn1 -- PMSM/LConn1
  Electrical Power/LConn1 -- +/RConn1
  -/RConn1 -- Electrical Power/LConn2 -- PMSM/RConn1
  Power/RConn2 -- PMSM/RConn2
  Torque Sensor/RConn1 -- R/RConn1
  Power/RConn1 -- Torque Sensor/LConn2

== system ssc_aircraft_elec_hybrid/Heater ==
  Conductive Heat Transfer : fl_lib/Thermal/Thermal Elements/Conductive Heat Transfer  thermal_type=foundation.enum.ConstantVariableTabulated.Constant  wall_geometry=foundation.enum.ConductionWallGeometry.Planar  area=1e-4 m^2  thickness=0.1 m  d_in=0.05 m  d_out=0.1 m  L=1 m  th_cond_min=10 W/(K*m)  th_cond=401 W/(m*K)  th_cond_TLU=[413, 401, 392, 383, 371, 357, 342] W/(K*m)  temp_TLU=[200, 273, 400, 600, 800, 1000, 1200] K  T_specify=off  T_priority=None  T=0 K  T_nominal_specify=off  T_nominal_value=1  T_nominal_unit=K  Q_specify=off  Q_priority=None  Q=0 J/s  Q_nominal_specify=off  Q_nominal_value=1  Q_nominal_unit=J/s
  Convective Heat Transfer : fl_lib/Thermal/Thermal Elements/Convective Heat Transfer  thermal_type=foundation.enum.constant_variable.constant  area=1e-4 m^2  heat_tr_coeff=20 W/(m^2 * K)  min_heat_tr_coeff=1e-3 W/(K*m^2)  T_specify=off  T_priority=None  T=0 K  T_nominal_specify=off  T_nominal_value=1  T_nominal_unit=K  Q_specify=off  Q_priority=None  Q=0 J/s  Q_nominal_specify=off  Q_nominal_value=1  Q_nominal_unit=J/s
  Electrical Power : Subsystem
  Thermal Resistor : fl_lib/Electrical/Electrical Elements/Thermal Resistor  R0=1 Ohm  T0=25 degC  alpha=5e-5 1/K  tc=10 s  K_d=1e-3 W/K  T_specify=on  T_priority=High  T=300 K  T_nominal_specify=off  T_nominal_value=1  T_nominal_unit=K
      settings: InternalSimscapePortConfiguration="{\"Bottom\":[],\"Left\":[{\"id\":\"H\",\"label\":\"H\",\"type\":\"foundation.thermal.thermal\"},{\"id\":\"p\",\"label\":\"+\",\"type\":\"foundation.electrical.electrical\"}],\"Right\":[{\"id\":\"n\",\"label\":\"-\",\"type\":\"foundation.electrical.electrical\"}],\"Top\":[]}"
  Thermal Mass : fl_lib/Thermal/Thermal Elements/Thermal Mass  mass_type=foundation.enum.constant_variable.constant  mass=1 kg  sp_heat=447 J/kg/K  mass_min=1e-6 kg  num_ports=foundation.enum.numPorts2.one  m_specify=off  m_priority=High  m=1 kg  m_nominal_specify=off  m_nominal_value=1  m_nominal_unit=kg  T_specify=on  T_priority=High  T=300 K  T_nominal_specify=off  T_nominal_value=1  T_nominal_unit=K  Q_specify=off  Q_priority=None  Q=0 J/s  Q_nominal_specify=off  Q_nominal_value=1  Q_nominal_unit=J/s
  Thermal Reference : fl_lib/Thermal/Thermal Elements/Thermal Reference
  + : PMIOPort  Side=Left
  - : PMIOPort  Port=2  Side=Left
  connections:
  Electrical Power/RConn1 -- Thermal Resistor/LConn2
  Convective Heat Transfer/LConn1 -- Thermal Mass/LConn1 -- Conductive Heat Transfer/RConn1
  Thermal Resistor/LConn1 -- Conductive Heat Transfer/LConn1
  Convective Heat Transfer/RConn1 -- Thermal Reference/LConn1
  -/RConn1 -- Electrical Power/LConn2 -- Thermal Resistor/RConn1
  Electrical Power/LConn1 -- +/RConn1

== system ssc_aircraft_elec_hybrid/Lamp ==
  Electrical Power : Subsystem
  Resistor : fl_lib/Electrical/Electrical Elements/Resistor  R=1 Ohm  i_specify=off  i_priority=None  i=0 A  i_nominal_specify=off  i_nominal_value=1  i_nominal_unit=A  v_specify=off  v_priority=None  v=0 V  v_nominal_specify=off  v_nominal_value=1  v_nominal_unit=V
  + : PMIOPort  Side=Left
  - : PMIOPort  Port=2  Side=Left
  connections:
  -/RConn1 -- Resistor/RConn1 -- Electrical Power/LConn2
  Resistor/LConn1 -- Electrical Power/RConn1
  Electrical Power/LConn1 -- +/RConn1
